simulink model "Interior_Light_Control"  (R2025a)
settings: Solver=VariableStepAuto  StartTime=0.0  StopTime=10.0  RelTol=1e-3
settings Model: Creator=nikul  LastModifiedBy=nikul

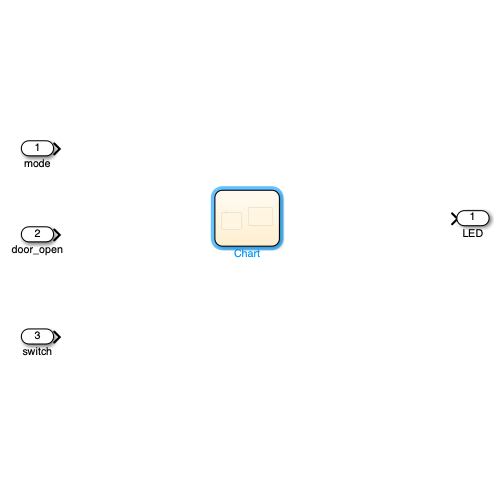
[thumbnail: Simulink's stored preview of the top-level diagram]
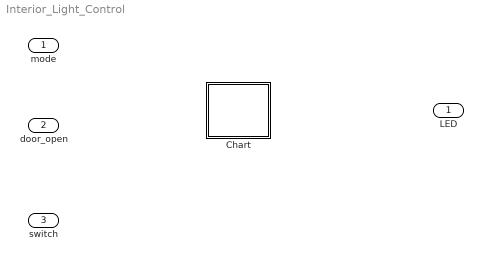
== system Interior_Light_Control ==
  mode : Inport
  door_open : Inport  Port=2
  switch : Inport  Port=3
  Chart : Stateflow chart  TreatAsAtomicUnit=on
  LED : Outport

== stateflow chart Interior_Light_Control/Chart ==
  state Manual_Mode
    if switch == 1
    LED = 1;
    else
    LED = 0;
    end
  state Auto_Mode
    if door_open == 1
    LED = 1;
    else
    LED = 0;
    end
  (default) -> Auto_Mode
